simulink model "ideal_block_diagram"  (R2024b)
settings: Solver=VariableStepAuto  StartTime=0.0  StopTime=10.0  RelTol=1e-3
libraries: autolibbldc x1
settings Model: Creator=jarre  LastModifiedBy=jarre

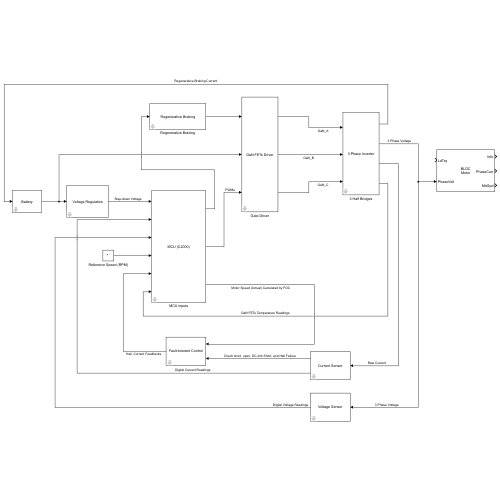
[thumbnail: Simulink's stored preview of the top-level diagram]
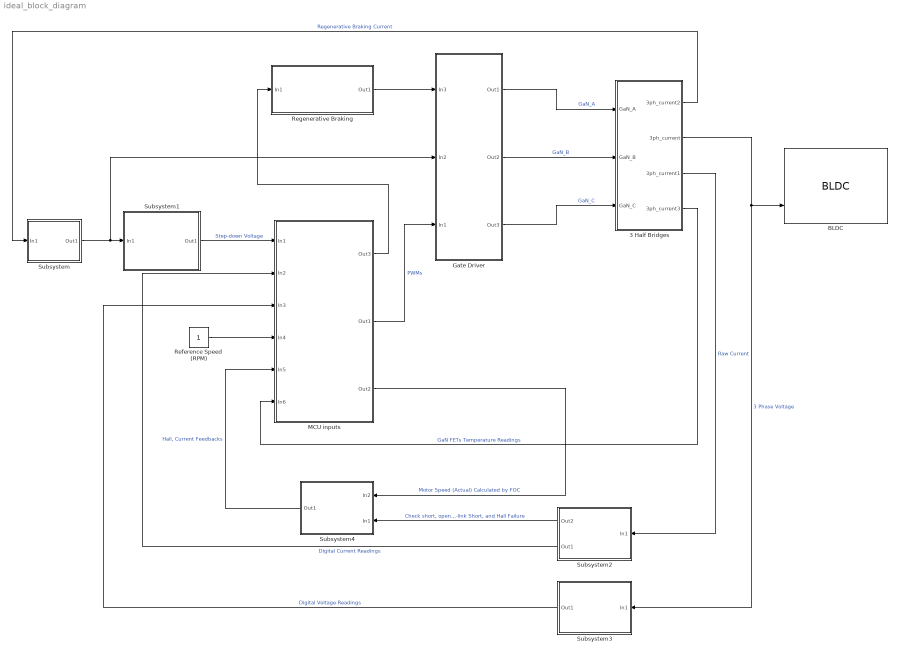
== system ideal_block_diagram ==
  3 Half Bridges : Subsystem
      mask Display: disp('3 Phase Inverter');
  BLDC : autolibbldc/BLDC  VariantControl=pmsmVariant==pmsmEnum.TorqueInput  MechInput=Torque  SimType=Continuous  BlockSampleTime=25e-6  p=4  Rs=0.36  Ld=2e-4  Lq=2e-4  Lambda=0.0064  J=7.0616e-06  B=2.6369e-06  F=0  Id_init=0  Iq_init=0  Th_init=0  Omega_init=0  RefBlkName='autolibbldc/BLDC'  aMode=5
      settings: LibrarySourceBlock=mcblib/Electrical Systems/Motors/BLDC
  Gate Driver : Subsystem
      mask Display: disp('GaN FETs Driver');
  MCU inputs : Subsystem
      mask Display: disp('MCU (C2000)');
  Reference Speed (RPM) : Constant
  Regenerative Braking : Subsystem
      mask Display: disp('Regenerative Braking');
  Subsystem : Subsystem
      mask Display: disp('Battery');
  Subsystem1 : Subsystem
      mask Display: disp('Voltage Regulation');
  Subsystem2 : Subsystem
      mask Display: disp('Current Sensor');
  Subsystem3 : Subsystem
      mask Display: disp('Voltage Sensor');
  Subsystem4 : Subsystem
      mask Display: disp('Fault-tolerant Control');
  wires:
  Gate Driver/1(Out1) -> 3 Half Bridges/1(GaN_A)  "GaN_A"
  Gate Driver/2(Out2) -> 3 Half Bridges/2(GaN_B)  "GaN_B"
  Gate Driver/3(Out3) -> 3 Half Bridges/3(GaN_C)  "GaN_C"
  MCU inputs/2(Out1) -> Gate Driver/3(In1)  "PWMs"
  3 Half Bridges/2(3ph_current) -> Subsystem3/1(In1), BLDC/2  "3 Phase Voltage"
  Subsystem1/1(Out1) -> MCU inputs/1(In1)  "Step-down Voltage"
  3 Half Bridges/3(3ph_current1) -> Subsystem2/1(In1)  "Raw Current"
  Subsystem2/2(Out1) -> MCU inputs/2(In2)  "Digital Current Readings"
  Subsystem3/1(Out1) -> MCU inputs/3(In3)  "Digital Voltage Readings"
  Reference Speed (RPM)/1 -> MCU inputs/4(In4)
  Regenerative Braking/1(Out1) -> Gate Driver/1(In3)
  3 Half Bridges/1(3ph_current2) -> Subsystem/1(In1)  "Regenerative Braking Current"
  Subsystem2/1(Out2) -> Subsystem4/2(In1)  "Check short, open, DC-link Short, and Hall Failure"
  Subsystem4/1(Out1) -> MCU inputs/5(In5)  "Hall, Current Feedbacks"
  3 Half Bridges/4(3ph_current3) -> MCU inputs/6(In6)  "GaN FETs Temperature Readings"
  MCU inputs/3(Out2) -> Subsystem4/1(In2)  "Motor Speed (Actual) Calculated by FOC"
  Subsystem/1(Out1) -> Gate Driver/2(In2), Subsystem1/1(In1)
  MCU inputs/1(Out3) -> Regenerative Braking/1(In1)

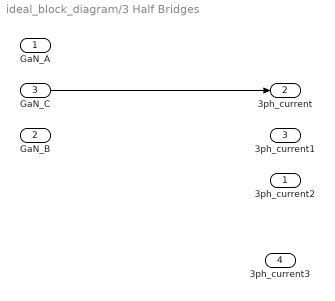
== system ideal_block_diagram/3 Half Bridges ==
  GaN_A : Inport
  GaN_B : Inport  Port=2
  GaN_C : Inport  Port=3
  3ph_current2 : Outport
  3ph_current : Outport  Port=2
  3ph_current1 : Outport  Port=3
  3ph_current3 : Outport  Port=4
  wires:
  GaN_C/1 -> 3ph_current/1

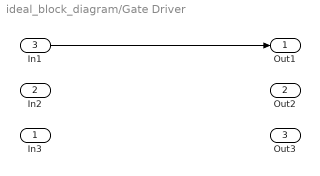
== system ideal_block_diagram/Gate Driver ==
  In3 : Inport
  In2 : Inport  Port=2
  In1 : Inport  Port=3
  Out1 : Outport
  Out2 : Outport  Port=2
  Out3 : Outport  Port=3
  wires:
  In1/1 -> Out1/1

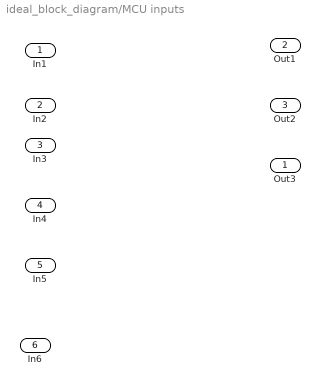
== system ideal_block_diagram/MCU inputs ==
  In1 : Inport
  In2 : Inport  Port=2
  In3 : Inport  Port=3
  In4 : Inport  Port=4
  In5 : Inport  Port=5
  In6 : Inport  Port=6
  Out3 : Outport
  Out1 : Outport  Port=2
  Out2 : Outport  Port=3

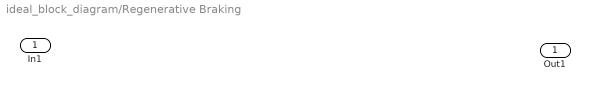
== system ideal_block_diagram/Regenerative Braking ==
  In1 : Inport
  Out1 : Outport

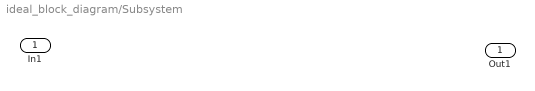
== system ideal_block_diagram/Subsystem ==
  In1 : Inport
  Out1 : Outport

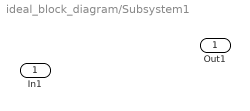
== system ideal_block_diagram/Subsystem1 ==
  In1 : Inport
  Out1 : Outport

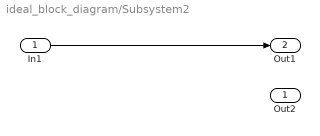
== system ideal_block_diagram/Subsystem2 ==
  In1 : Inport
  Out2 : Outport
  Out1 : Outport  Port=2
  wires:
  In1/1 -> Out1/1

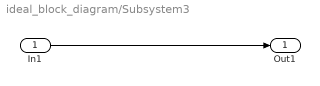
== system ideal_block_diagram/Subsystem3 ==
  In1 : Inport
  Out1 : Outport
  wires:
  In1/1 -> Out1/1

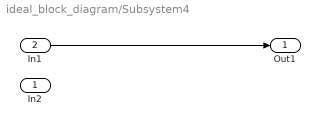
== system ideal_block_diagram/Subsystem4 ==
  In2 : Inport
  In1 : Inport  Port=2
  Out1 : Outport
  wires:
  In1/1 -> Out1/1
